simulink model "cruise_windup_PI_AW"  (R2026b)
settings: Solver=FixedStepDiscrete  StopTime=120  FixedStep=0.01
model workspace (MAT data in the model file):
  grade_input = [0 0.01 0.02 0.03 0.04 0.05 0.06 0.07 0.08 0.09 0.1 0.11 ... (24002 elements, 12001x2)]
  limit_input = [0 0.01 0.02 0.03 0.04 0.05 0.06 0.07 0.08 0.09 0.1 0.11 ... (24002 elements, 12001x2)]
  ref_input = [0 0.01 0.02 0.03 0.04 0.05 0.06 0.07 0.08 0.09 0.1 0.11 ... (24002 elements, 12001x2)]
settings Model: Creator=volkanakyazici  LastModifiedBy=volkanakyazici

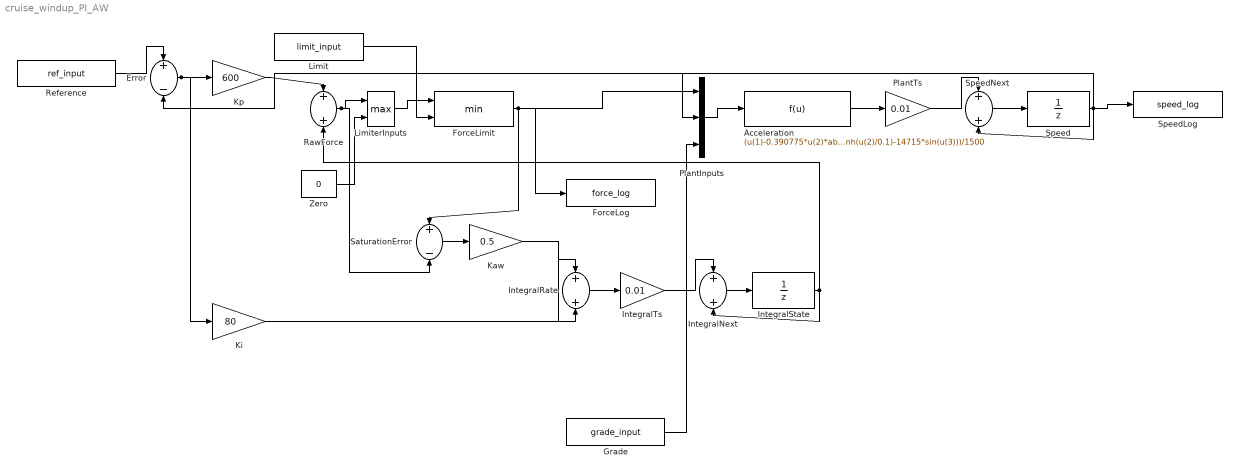
== system cruise_windup_PI_AW ==
  Acceleration : Fcn  Expr=(u(1)-0.390775*u(2)*abs(u(2))-176.58*cos(u(3))*tanh(u(2)/0.1)-14715*sin(u(3)))/1500
  Error : Sum  Inputs=+-
  ForceLimit : MinMax  Inputs=2
  ForceLog : ToWorkspace  VariableName=force_log  SaveFormat=Timeseries  SampleTime=-1
  Grade : FromWorkspace  VariableName=grade_input  SampleTime=0.01  Interpolate=off  OutputAfterFinalValue=Holding final value
  IntegralNext : Sum
  IntegralRate : Sum
  IntegralState : UnitDelay  SampleTime=0.01
  IntegralTs : Gain  Gain=0.01
  Kaw : Gain  Gain=0.5
  Ki : Gain  Gain=80
  Kp : Gain  Gain=600
  Limit : FromWorkspace  VariableName=limit_input  SampleTime=0.01  Interpolate=off  OutputAfterFinalValue=Holding final value
  LimiterInputs : MinMax  Function=max  Inputs=2
  PlantInputs : Mux  Inputs=3
  PlantTs : Gain  Gain=0.01
  RawForce : Sum
  Reference : FromWorkspace  VariableName=ref_input  SampleTime=0.01  Interpolate=off  OutputAfterFinalValue=Holding final value
  SaturationError : Sum  Inputs=+-
  Speed : UnitDelay  InitialCondition=15  SampleTime=0.01
  SpeedLog : ToWorkspace  VariableName=speed_log  SaveFormat=Timeseries  SampleTime=-1
  SpeedNext : Sum
  Zero : Constant  Value=0
  wires:
  Reference/1 -> Error/1
  Speed/1 -> Error/2, PlantInputs/2, SpeedNext/2, SpeedLog/1
  Error/1 -> Kp/1, Ki/1
  Kp/1 -> RawForce/1
  IntegralState/1 -> RawForce/2, IntegralNext/2
  RawForce/1 -> LimiterInputs/1, SaturationError/2
  Zero/1 -> LimiterInputs/2
  LimiterInputs/1 -> ForceLimit/1
  Limit/1 -> ForceLimit/2
  ForceLimit/1 -> SaturationError/1, PlantInputs/1, ForceLog/1
  SaturationError/1 -> Kaw/1
  Ki/1 -> IntegralRate/1
  Kaw/1 -> IntegralRate/2
  IntegralRate/1 -> IntegralTs/1
  IntegralTs/1 -> IntegralNext/1
  IntegralNext/1 -> IntegralState/1
  Grade/1 -> PlantInputs/3
  PlantInputs/1 -> Acceleration/1
  Acceleration/1 -> PlantTs/1
  PlantTs/1 -> SpeedNext/1
  SpeedNext/1 -> Speed/1
